simulink model "AGV_MISSION"  (R2025a)
settings: Solver=FixedStepDiscrete  StartTime=0.0  StopTime=P.agv.Tend  FixedStep=P.ctrl.Ts  RelTol=1e-3
undefined symbols (not defined in the file or in its folder): DiscIntNeverNeededParam, P
libraries: simulink x1
settings Model: Creator=USER  LastModifiedBy=USER
settings DataIOCC: SaveOutput=off  SignalLogging=off  SaveTime=off

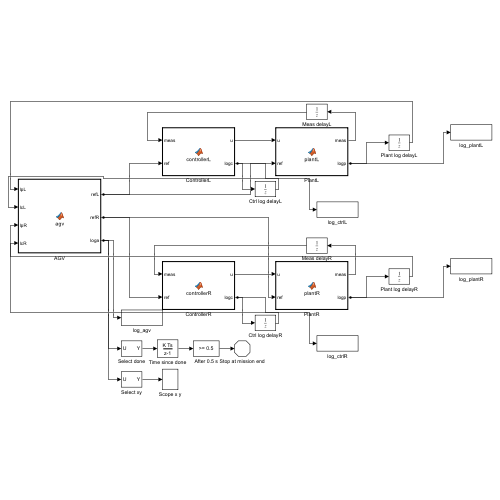
[thumbnail: Simulink's stored preview of the top-level diagram]
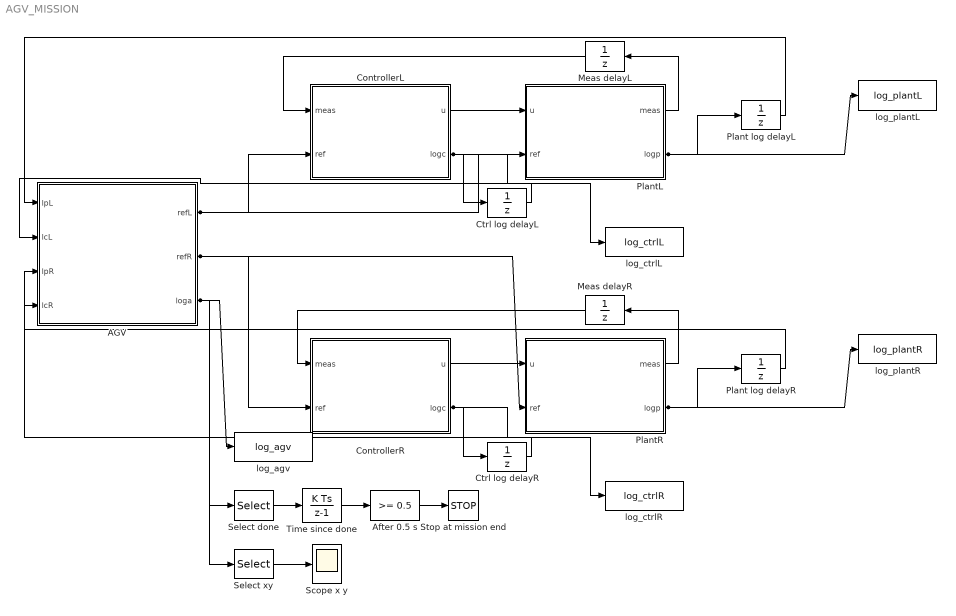
== system AGV_MISSION ==
  AGV : MATLAB Function  TreatAsAtomicUnit=on
  After 0.5 s : simulink/Logic and Bit Operations/Compare To Constant  relop=>=  const=0.5  OutDataTypeStr=boolean
  ControllerL : MATLAB Function  TreatAsAtomicUnit=on
  ControllerR : MATLAB Function  TreatAsAtomicUnit=on
  Ctrl log delayL : UnitDelay  InitialCondition=zeros(16,1)  SampleTime=P.ctrl.Ts  HasFrameUpgradeWarning=on
  Ctrl log delayR : UnitDelay  InitialCondition=zeros(16,1)  SampleTime=P.ctrl.Ts  HasFrameUpgradeWarning=on
  Meas delayL : UnitDelay  InitialCondition=zeros(4,1)  SampleTime=P.ctrl.Ts  HasFrameUpgradeWarning=on
  Meas delayR : UnitDelay  InitialCondition=zeros(4,1)  SampleTime=P.ctrl.Ts  HasFrameUpgradeWarning=on
  Plant log delayL : UnitDelay  InitialCondition=zeros(23,1)  SampleTime=P.ctrl.Ts  HasFrameUpgradeWarning=on
  Plant log delayR : UnitDelay  InitialCondition=zeros(23,1)  SampleTime=P.ctrl.Ts  HasFrameUpgradeWarning=on
  PlantL : MATLAB Function  TreatAsAtomicUnit=on
  PlantR : MATLAB Function  TreatAsAtomicUnit=on
  Scope x y : Scope
  Select done : Selector  InputPortWidth=16  IndexOptions=Index vector (dialog)  Indices=13  OutputSizes=1
  Select xy : Selector  InputPortWidth=16  IndexOptions=Index vector (dialog)  Indices=[1 2]  OutputSizes=1
  Stop at mission end : Stop
  Time since done : DiscreteIntegrator  SampleTime=P.ctrl.Ts  ICPrevOutput=DiscIntNeverNeededParam  ICPrevScaledInput=DiscIntNeverNeededParam
  log_agv : ToWorkspace  VariableName=log_agv  SaveFormat=Structure With Time  SampleTime=-1
      settings: Decimation=P.agv.log_decim
  log_ctrlL : ToWorkspace  VariableName=log_ctrlL  SaveFormat=Structure With Time  SampleTime=-1
      settings: Decimation=P.agv.log_decim
  log_ctrlR : ToWorkspace  VariableName=log_ctrlR  SaveFormat=Structure With Time  SampleTime=-1
      settings: Decimation=P.agv.log_decim
  log_plantL : ToWorkspace  VariableName=log_plantL  SaveFormat=Structure With Time  SampleTime=-1
      settings: Decimation=P.agv.log_decim
  log_plantR : ToWorkspace  VariableName=log_plantR  SaveFormat=Structure With Time  SampleTime=-1
      settings: Decimation=P.agv.log_decim
  wires:
  AGV/1(refL) -> ControllerL/2(ref), PlantL/2(ref)
  ControllerL/1(u) -> PlantL/1(u)
  PlantL/1(meas) -> Meas delayL/1
  Meas delayL/1 -> ControllerL/1(meas)
  PlantL/2(logp) -> Plant log delayL/1, log_plantL/1
  ControllerL/2(logc) -> Ctrl log delayL/1, log_ctrlL/1
  AGV/2(refR) -> ControllerR/2(ref), PlantR/2(ref)
  ControllerR/1(u) -> PlantR/1(u)
  PlantR/1(meas) -> Meas delayR/1
  Meas delayR/1 -> ControllerR/1(meas)
  PlantR/2(logp) -> Plant log delayR/1, log_plantR/1
  ControllerR/2(logc) -> Ctrl log delayR/1, log_ctrlR/1
  Plant log delayL/1 -> AGV/1(lpL)
  Ctrl log delayL/1 -> AGV/2(lcL)
  Plant log delayR/1 -> AGV/3(lpR)
  Ctrl log delayR/1 -> AGV/4(lcR)
  AGV/3(loga) -> log_agv/1, Select done/1, Select xy/1
  Select done/1 -> Time since done/1
  Time since done/1 -> After 0.5 s/1
  After 0.5 s/1 -> Stop at mission end/1
  Select xy/1 -> Scope x y/1

== matlab function AGV_MISSION/ControllerL ==
  data: meas input; u output; ref input; logc output; P parameter
function [u, logc] = controllerL(meas, ref, P)
%#codegen
persistent st
if isempty(st)
    st = ctrl_init(P);
end
[u, logc, st] = ctrl_step(st, meas, ref, P);

== matlab function AGV_MISSION/AGV ==
  data: lpL input; refL output; lcL input; lpR input; lcR input; refR output; loga output; P parameter
function [refL, refR, loga] = agv(lpL, lcL, lpR, lcR, P)
%#codegen
% Robot kinematics, pure pursuit, mission and fault supervisor (agv/agv_step.m)
persistent ast
if isempty(ast)
    ast = agv_init(P);
end
[refL, refR, loga, ast] = agv_step(ast, lpL, lcL, lpR, lcR, P);

== matlab function AGV_MISSION/PlantL ==
  data: u input; meas output; ref input; logp output; P parameter
function [meas, logp] = plantL(u, ref, P)
%#codegen
persistent pst
if isempty(pst)
    pst = plant_init(P);
end
[meas, logp, pst] = plant_step(pst, u, ref, P);

== matlab function AGV_MISSION/ControllerR ==
  data: meas input; u output; ref input; logc output; P parameter
function [u, logc] = controllerR(meas, ref, P)
%#codegen
persistent st
if isempty(st)
    st = ctrl_init(P);
end
[u, logc, st] = ctrl_step(st, meas, ref, P);

== matlab function AGV_MISSION/PlantR ==
  data: u input; meas output; ref input; logp output; P parameter
function [meas, logp] = plantR(u, ref, P)
%#codegen
persistent pst
if isempty(pst)
    pst = plant_init(P);
end
[meas, logp, pst] = plant_step(pst, u, ref, P);
